simulink model "cartpole"  (R2026b)
settings: Solver=ode4  StopTime=15  FixedStep=0.01
model workspace (MAT data in the model file):
  cfg.M = 1
  cfg.m = 0.1
  cfg.ell = 0.5
  cfg.g = 9.81
  cfg.h = 0.01
  cfg.forceLimit = 10
  cfg.trackLimit = 2.4
  cfg.angleLimit = 1.0471975512
  cfg.initial = [0.25; 0; 0.13962634016; 0]
  cfg.bias = 0
  cfg.ki = 1.46788990826
  cfg.kp = 4.28134556575
  cfg.kd = 4.76390876189
  cfg.D = 7.98195438094
  cfg.K = 36.4316727829
settings Model: Creator=Phuc Minh Quan  LastModifiedBy=Phuc Minh Quan

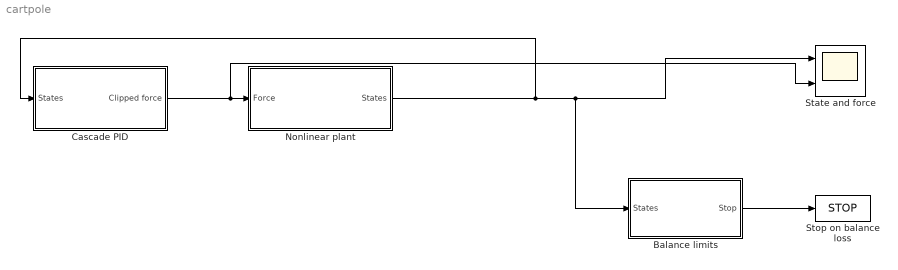
== system cartpole ==
  Balance limits : Subsystem
  Cascade PID : Subsystem
  Nonlinear plant : Subsystem
  State and force : Scope  NumInputPorts=2
      settings: ActiveDisplayYMinimum=-5.4342933497206944  ActiveDisplayYMaximum=8.6344412375254631
  Stop on balance loss : Stop
  wires:
  Cascade PID/1(Clipped force) -> Nonlinear plant/1(Force), State and force/2
  Nonlinear plant/1(States) -> Balance limits/1(States), State and force/1, Cascade PID/1(States)
  Balance limits/1(Stop) -> Stop on balance loss/1

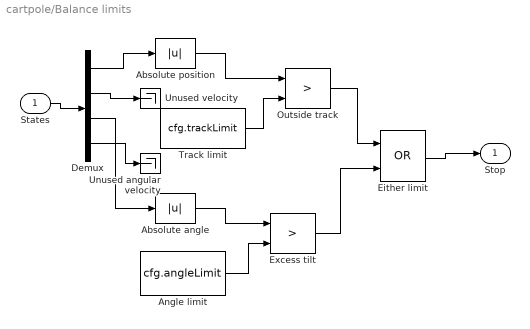
== system cartpole/Balance limits ==
  States : Inport
  Absolute angle : Abs  SaturateOnIntegerOverflow=off
  Absolute position : Abs  SaturateOnIntegerOverflow=off
  Angle limit : Constant  Value=cfg.angleLimit
  Demux : Demux
  Either limit : Logic  Operator=OR  AllPortsSameDT=off  OutDataTypeStr=boolean
  Excess tilt : RelationalOperator  Operator=>  OutDataTypeStr=boolean  RndMeth=Simplest  InputSameDT=off
  Outside track : RelationalOperator  Operator=>  OutDataTypeStr=boolean  RndMeth=Simplest  InputSameDT=off
  Track limit : Constant  Value=cfg.trackLimit
  Unused angular velocity : Terminator
  Unused velocity : Terminator
  Stop : Outport
  wires:
  States/1 -> Demux/1
  Demux/1 -> Absolute position/1
  Demux/2 -> Unused velocity/1
  Demux/3 -> Absolute angle/1
  Demux/4 -> Unused angular velocity/1
  Absolute position/1 -> Outside track/1
  Track limit/1 -> Outside track/2
  Absolute angle/1 -> Excess tilt/1
  Angle limit/1 -> Excess tilt/2
  Outside track/1 -> Either limit/1
  Excess tilt/1 -> Either limit/2
  Either limit/1 -> Stop/1

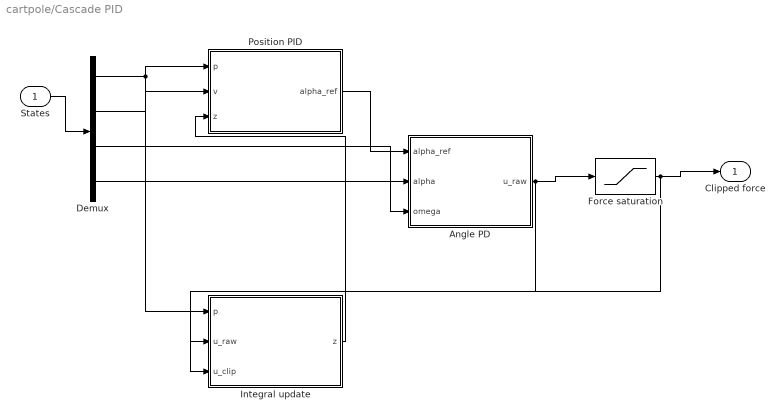
== system cartpole/Cascade PID ==
  States : Inport
  Angle PD : Subsystem
  Demux : Demux
  Force saturation : Saturate  UpperLimit=cfg.forceLimit  LowerLimit=-cfg.forceLimit
  Integral update : Subsystem
  Position PID : Subsystem
  Clipped force : Outport
  wires:
  States/1 -> Demux/1
  Demux/1 -> Position PID/1(p), Integral update/1(p)
  Demux/2 -> Position PID/2(v)
  Integral update/1(z) -> Position PID/3(z)
  Position PID/1(alpha_ref) -> Angle PD/1(alpha_ref)
  Demux/3 -> Angle PD/2(alpha)
  Demux/4 -> Angle PD/3(omega)
  Angle PD/1(u_raw) -> Force saturation/1, Integral update/2(u_raw)
  Force saturation/1 -> Clipped force/1, Integral update/3(u_clip)

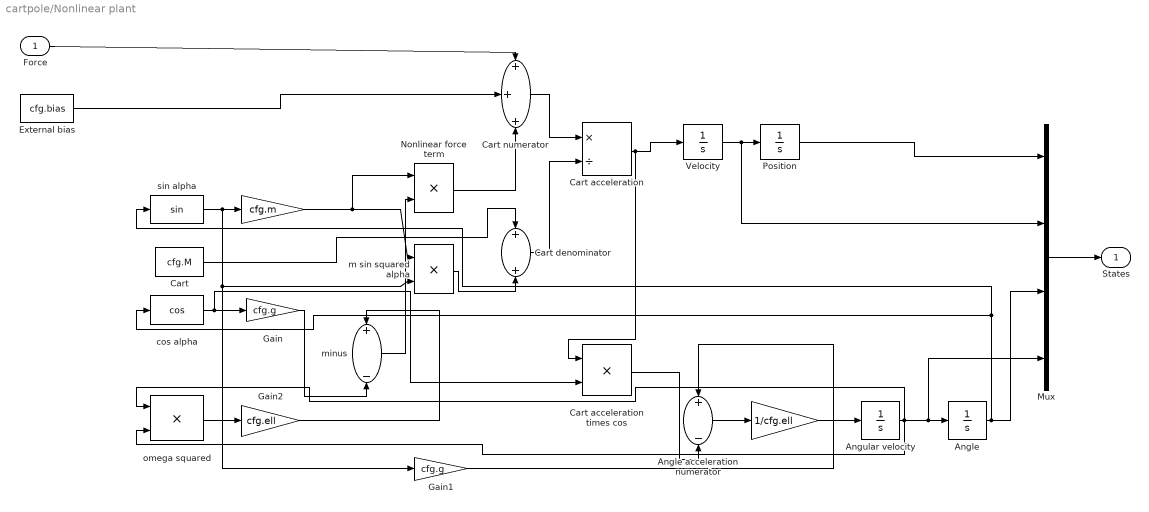
== system cartpole/Nonlinear plant ==
  Force : Inport
  " " : Gain  Gain=cfg.m
  "  " : Gain  Gain=1/cfg.ell
  Angle : Integrator  InitialCondition=cfg.initial(3)
  Angle acceleration numerator : Sum  Inputs=+-
  Angular velocity : Integrator  InitialCondition=cfg.initial(4)
  "Cart " : Constant  Value=cfg.M
  Cart acceleration : Product  Inputs=*/
  Cart acceleration times cos : Product  Inputs=**
  Cart denominator : Sum
  Cart numerator : Sum  Inputs=+++
  External bias : Constant  Value=cfg.bias
  Gain : Gain  Gain=cfg.g
  Gain1 : Gain  Gain=cfg.g
  Gain2 : Gain  Gain=cfg.ell
  Mux : Mux
  Nonlinear force term : Product  Inputs=**
  Position : Integrator  InitialCondition=cfg.initial(1)
  Velocity : Integrator  InitialCondition=cfg.initial(2)
  cos alpha : Trigonometry  Operator=cos
  m sin squared alpha : Product  Inputs=**
  minus : Sum  Inputs=+-
  omega squared : Product  Inputs=**
  sin alpha : Trigonometry
  States : Outport
  wires:
  Angle/1 -> sin alpha/1, cos alpha/1, Mux/3
  Angular velocity/1 -> Angle/1, Mux/4, omega squared/1, omega squared/2
  omega squared/1 -> Gain2/1
  cos alpha/1 -> Gain/1, Cart acceleration times cos/2
  Gain2/1 -> minus/1
  Gain/1 -> minus/2
  sin alpha/1 -> Gain1/1, m sin squared alpha/2, " "/1
  " "/1 -> Nonlinear force term/1, m sin squared alpha/1
  minus/1 -> Nonlinear force term/2
  Force/1 -> Cart numerator/1
  External bias/1 -> Cart numerator/2
  Nonlinear force term/1 -> Cart numerator/3
  "Cart "/1 -> Cart denominator/1
  m sin squared alpha/1 -> Cart denominator/2
  Cart numerator/1 -> Cart acceleration/1
  Cart denominator/1 -> Cart acceleration/2
  Cart acceleration/1 -> Velocity/1, Cart acceleration times cos/1
  Velocity/1 -> Position/1, Mux/2
  Gain1/1 -> Angle acceleration numerator/1
  Cart acceleration times cos/1 -> Angle acceleration numerator/2
  Angle acceleration numerator/1 -> "  "/1
  "  "/1 -> Angular velocity/1
  Position/1 -> Mux/1
  Mux/1 -> States/1

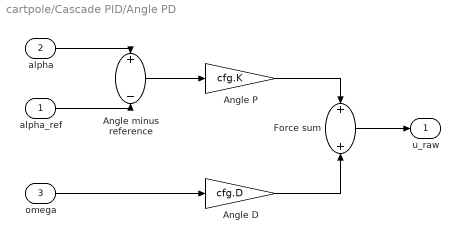
== system cartpole/Cascade PID/Angle PD ==
  alpha_ref : Inport
  alpha : Inport  Port=2
  omega : Inport  Port=3
  Angle D : Gain  Gain=cfg.D
  Angle P : Gain  Gain=cfg.K
  Angle minus reference : Sum  Inputs=+-
  Force sum : Sum
  u_raw : Outport
  wires:
  alpha/1 -> Angle minus reference/1
  alpha_ref/1 -> Angle minus reference/2
  Angle minus reference/1 -> Angle P/1
  omega/1 -> Angle D/1
  Angle P/1 -> Force sum/1
  Angle D/1 -> Force sum/2
  Force sum/1 -> u_raw/1

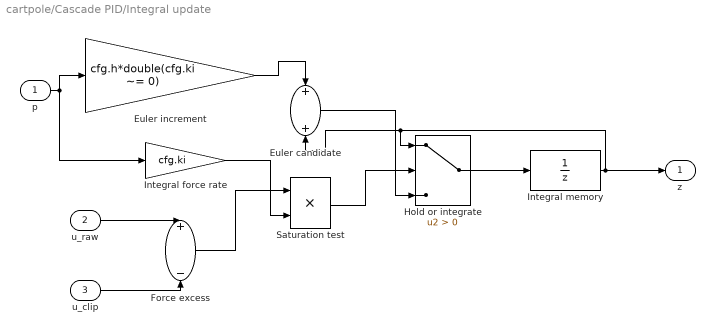
== system cartpole/Cascade PID/Integral update ==
  p : Inport
  u_raw : Inport  Port=2
  u_clip : Inport  Port=3
  Euler candidate : Sum
  Euler increment : Gain  Gain=cfg.h*double(cfg.ki ~= 0)
  Force excess : Sum  Inputs=+-
  Hold or integrate : Switch  Criteria=u2 > Threshold  SaturateOnIntegerOverflow=off  InputSameDT=off
  Integral force rate : Gain  Gain=cfg.ki
  Integral memory : UnitDelay  SampleTime=cfg.h
  Saturation test : Product  Inputs=**
  z : Outport
  wires:
  p/1 -> Integral force rate/1, Euler increment/1
  u_raw/1 -> Force excess/1
  u_clip/1 -> Force excess/2
  Force excess/1 -> Saturation test/1
  Integral force rate/1 -> Saturation test/2
  Euler increment/1 -> Euler candidate/1
  Integral memory/1 -> Euler candidate/2, Hold or integrate/1, z/1
  Saturation test/1 -> Hold or integrate/2
  Euler candidate/1 -> Hold or integrate/3
  Hold or integrate/1 -> Integral memory/1

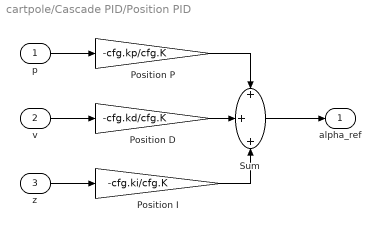
== system cartpole/Cascade PID/Position PID ==
  p : Inport
  v : Inport  Port=2
  z : Inport  Port=3
  Position D : Gain  Gain=-cfg.kd/cfg.K
  Position I : Gain  Gain=-cfg.ki/cfg.K
  Position P : Gain  Gain=-cfg.kp/cfg.K
  Sum : Sum  Inputs=+++
  alpha_ref : Outport
  wires:
  p/1 -> Position P/1
  v/1 -> Position D/1
  z/1 -> Position I/1
  Position P/1 -> Sum/1
  Position D/1 -> Sum/2
  Position I/1 -> Sum/3
  Sum/1 -> alpha_ref/1
